simulink model "PenduloQUBE"  (R2025b)
settings: Solver=ode4  StartTime=0.0  StopTime=T_final  FixedStep=0.001  RelTol=1e-3
values from neighbouring files (symbols this model uses):
  alpha0 = deg2rad(2)    [entrenamiento.m]    (also in evaluar.m = deg2rad((rand() - 0.5) * 20))
  alpha_dot0 = 0    [entrenamiento.m]    (also in evaluar.m = deg2rad((rand() - 0.5) * 120))
  theta0 = 0    [entrenamiento.m]    (also in evaluar.m = deg2rad((rand() - 0.5) * 60))
  theta_dot0 = 0    [entrenamiento.m]    (also in evaluar.m = deg2rad((rand() - 0.5) * 300))
  Ts = 0.01    [entrenamiento.m]    (also in evaluar.m)
libraries: rllib x1
settings Model: Creator=leogo  LastModifiedBy=leogo

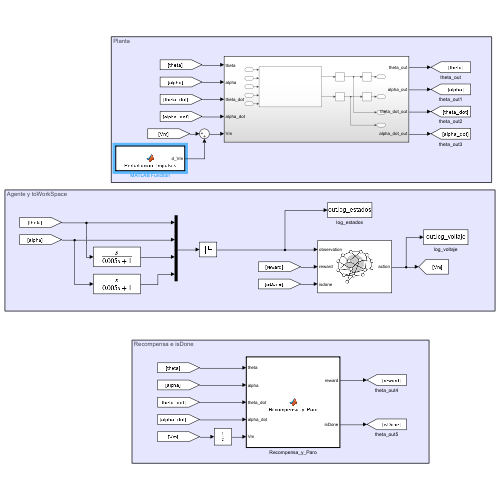
[thumbnail: Simulink's stored preview of the top-level diagram]
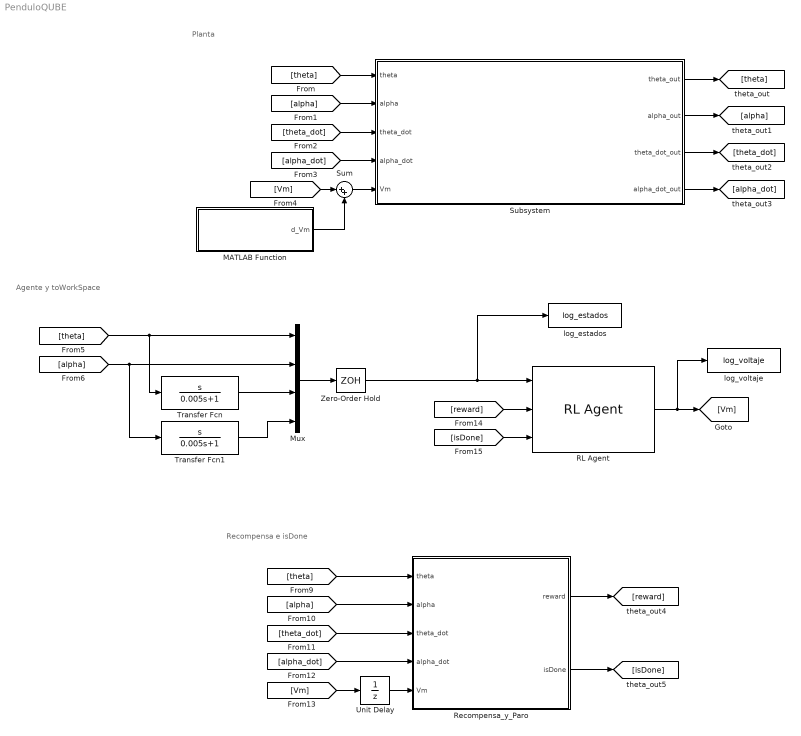
== system PenduloQUBE ==
  note: Agente y toWorkSpace
  note: Recompensa e isDone
  note: Planta
  MATLAB Function : MATLAB Function  TreatAsAtomicUnit=on  SystemSampleTime=0.1
  Mux : Mux
  RL Agent : rllib/RL Agent  Agent=agente  ExternalActionAsInput=off  ProvideLastAction=off  ProvideCumRwd=off  TreatAsDirectFeedthrough=on  UseStrictObservationDataTypes=off
  Recompensa_y_Paro : MATLAB Function  TreatAsAtomicUnit=on
  Subsystem : Subsystem
  Sum : Sum  Inputs=|++
  Transfer Fcn : TransferFcn  Numerator=[1 0]  Denominator=[0.005 1]
  Transfer Fcn1 : TransferFcn  Numerator=[1 0]  Denominator=[0.005 1]
  Unit Delay : UnitDelay  SampleTime=-1  HasFrameUpgradeWarning=on
  Zero-Order Hold : ZeroOrderHold  SampleTime=Ts
  log_estados : ToWorkspace  VariableName=log_estados  SaveFormat=Timeseries  SampleTime=-1
  log_voltaje : ToWorkspace  VariableName=log_voltaje  SaveFormat=Timeseries  SampleTime=-1
  wires:
  Mux/1 -> Zero-Order Hold/1
  Zero-Order Hold/1 -> log_estados/1, RL Agent/1
  Subsystem/1(theta_out) -> [theta]
  Subsystem/2(alpha_out) -> [alpha]
  Subsystem/3(theta_dot_out) -> [theta_dot]
  Subsystem/4(alpha_dot_out) -> [alpha_dot]
  [theta] -> Subsystem/1(theta)
  [alpha] -> Subsystem/2(alpha)
  [theta_dot] -> Subsystem/3(theta_dot)
  [alpha_dot] -> Subsystem/4(alpha_dot)
  RL Agent/1 -> log_voltaje/1, [Vm]
  [theta] -> Transfer Fcn/1, Mux/1
  [alpha] -> Mux/2, Transfer Fcn1/1
  Transfer Fcn/1 -> Mux/3
  Transfer Fcn1/1 -> Mux/4
  [theta] -> Recompensa_y_Paro/1(theta)
  [alpha] -> Recompensa_y_Paro/2(alpha)
  [theta_dot] -> Recompensa_y_Paro/3(theta_dot)
  [alpha_dot] -> Recompensa_y_Paro/4(alpha_dot)
  [Vm] -> Unit Delay/1
  Recompensa_y_Paro/1(reward) -> [reward]
  Recompensa_y_Paro/2(isDone) -> [isDone]
  [reward] -> RL Agent/2
  [isDone] -> RL Agent/3
  Unit Delay/1 -> Recompensa_y_Paro/5(Vm)
  Sum/1 -> Subsystem/5(Vm)
  [Vm] -> Sum/1
  MATLAB Function/1(d_Vm) -> Sum/2

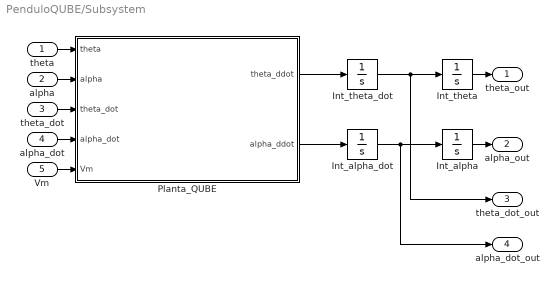
== system PenduloQUBE/Subsystem ==
  theta : Inport
  alpha : Inport  Port=2
  theta_dot : Inport  Port=3
  alpha_dot : Inport  Port=4
  Vm : Inport  Port=5
  Int_alpha : Integrator  InitialCondition=alpha0
  Int_alpha_dot : Integrator  InitialCondition=alpha_dot0
  Int_theta : Integrator  InitialCondition=theta0
  Int_theta_dot : Integrator  InitialCondition=theta_dot0
  Planta_QUBE : MATLAB Function  TreatAsAtomicUnit=on
  theta_out : Outport
  alpha_out : Outport  Port=2
  theta_dot_out : Outport  Port=3
  alpha_dot_out : Outport  Port=4
  wires:
  Planta_QUBE/2(alpha_ddot) -> Int_alpha_dot/1
  Int_alpha_dot/1 -> alpha_dot_out/1, Int_alpha/1
  theta_dot/1 -> Planta_QUBE/3(theta_dot)
  Int_theta/1 -> theta_out/1
  Int_theta_dot/1 -> theta_dot_out/1, Int_theta/1
  Planta_QUBE/1(theta_ddot) -> Int_theta_dot/1
  theta/1 -> Planta_QUBE/1(theta)
  alpha/1 -> Planta_QUBE/2(alpha)
  Vm/1 -> Planta_QUBE/5(Vm)
  alpha_dot/1 -> Planta_QUBE/4(alpha_dot)
  Int_alpha/1 -> alpha_out/1

== matlab function PenduloQUBE/Recompensa_y_Paro ==
  data: theta input; reward output; alpha input; theta_dot input; alpha_dot input; Vm input; isDone output
function [reward, isDone] = Recompensa_y_Paro(theta, alpha, theta_dot, alpha_dot, Vm)
    % =====================================================================
    % Función de Recompensa (Propuesta A) y Condición de Paro (isDone)
    % =====================================================================

    % 1. Límites de operación segura en radianes
    alpha_lim = deg2rad(15);  % +-15 grados para el péndulo (~0.2618 rad)
    theta_lim = deg2rad(90);  % +-90 grados para el brazo (~1.5708 rad)

    % 2. Evaluar condición de término (isDone como escalar booleano)
    fuera_de_rango = (abs(alpha) > alpha_lim) || (abs(theta) > theta_lim);
    isDone = boolean(fuera_de_rango);

    % 3. Cálculo de la recompensa
    if isDone
        % Castigo severo por dejar caer el péndulo o chocar el brazo
        reward = -100.0;
    else
        % Pesos de penalización cuadrática (Ecuación 5 del documento)
        q_alpha     = 10.0;   % Prioridad máxima: péndulo en 0 rad
        q_theta     = 4.0;    % Prioridad media: brazo centrado en 0 rad
        q_alpha_dot = 0.1;    % Amortiguamiento del péndulo
        q_theta_dot = 0.05;   % Amortiguamiento del brazo
        rho         = 0.02;  % Penalización de esfuerzo de voltaje (Vm)

        costo_cuadratico = q_alpha * (alpha^2) ...
                         + q_theta * (theta^2) ...
                         + q_alpha_dot * (alpha_dot^2) ...
                         + q_theta_dot * (theta_dot^2) ...
                         + rho * (Vm^2);

        % Bono de supervivencia (+1.0) menos el costo cuadrático, evita el
        % suicidio
        reward = 1.0 - costo_cuadratico;
    end
end

== matlab function PenduloQUBE/Subsystem/Planta_QUBE ==
  data: theta input; theta_ddot output; alpha input; theta_dot input; alpha_dot input; Vm input; alpha_ddot output
function [theta_ddot, alpha_ddot] = Planta_QUBE(theta, alpha, theta_dot, alpha_dot, Vm)
    % =====================================================================
    % Modelo Dinámico No Lineal del Quanser QUBE-Servo 3 (Péndulo Rotatorio)
    % α = 0 rad corresponde a la posición vertical invertida
    % =====================================================================

    % 1. Parámetros nominales (Cuadro 2 del documento)
    Rm = 8.4;       % Resistencia de armadura [Ohm]
    km = 0.042;     % Constante par / fuerza contraelectromotriz [N*m/A]
    mr = 0.095;     % Masa del brazo rotatorio [kg]
    Lr = 0.085;     % Longitud del brazo rotatorio [m]
    mp = 0.024;     % Masa del péndulo [kg]
    Lp = 0.129;     % Longitud total del péndulo [m]
    Dr = 0.0015;    % Amortiguamiento viscoso del brazo [N*m*s/rad]
    Dp = 0.0005;    % Amortiguamiento viscoso del péndulo [N*m*s/rad]
    g  = 9.81;      % Gravedad [m/s^2]

    % Momentos de inercia respecto al centro de masa
    Jr = (mr * Lr^2) / 12;
    Jp = (mp * Lp^2) / 12;

    % 2. Saturación de seguridad del voltaje del motor
    Vm_sat = max(min(Vm, 12.0), -12.0);

    % 3. Par electromecánico aplicado por el motor DC
    tau = (km * (Vm_sat - km * theta_dot)) / Rm;

    % 4. Matriz de masas/inercia acoplada M(alpha) * [theta_ddot; alpha_ddot] = RHS
    M11 = mp * Lr^2 + 0.25 * mp * Lp^2 - 0.25 * mp * Lp^2 * (cos(alpha)^2) + Jr;
    M12 = -0.5 * mp * Lp * Lr * cos(alpha);
    M21 = -0.5 * mp * Lp * Lr * cos(alpha);
    M22 = Jp + 0.25 * mp * Lp^2;

    % 5. Vector de términos no lineales (Coriolis, centrífugos, fricción y gravedad)
    RHS1 = tau - Dr * theta_dot ...
           - (0.5 * mp * Lp^2 * sin(alpha) * cos(alpha)) * theta_dot * alpha_dot ...
           - (0.5 * mp * Lp * Lr * sin(alpha)) * (alpha_dot^2);

    % Nota: El término de gravedad lleva signo positivo en RHS2 porque en alpha = 0 
    % (invertido) la gravedad empuja al péndulo alejándolo del equilibrio (inestable).
    RHS2 = -Dp * alpha_dot ...
           + (0.25 * mp * Lp^2 * cos(alpha) * sin(alpha)) * (theta_dot^2) ...
           + 0.5 * mp * Lp * g * sin(alpha);

    % 6. Solución por regla de Cramer (más rápida en Simulink que inv(M))
    detM = M11 * M22 - M12 * M21;
    theta_ddot = ( M22 * RHS1 - M12 * RHS2) / detM;
    alpha_ddot = (-M21 * RHS1 + M11 * RHS2) / detM;
end

== matlab function PenduloQUBE/MATLAB Function ==
  data: d_Vm output
function d_Vm = Perturbacion_Impulsos()
% Configurar Sample time del bloque en: 0.1 (100 ms por pulso)

p = rand();           % Probabilidad entre 0 y 1
r = 2 * rand() - 1;   % Valor aleatorio entre -1 y +1

if p < 0.10
    % 10% de las veces (1 empujón fuerte de 100 ms cada ~1 segundo):
    % Pulso severo de entre -5.5 V y +5.5 V (casi el 70% de la fuerza máxima del agente)
    d_Vm = 5.5 * r;
else
    % 90% del tiempo: Fricción/vibración base entre -0.5 V y +0.5 V
    d_Vm = 0.5 * r;
end
end
